simulink library "Yaw_Gearbox_Lib"  (R2025a)
settings: Solver=ode45  StartTime=0.0  StopTime=10.0  RelTol=1e-3  EnableMultiTasking=on
undefined symbols (not defined in the file): WT_Params
libraries: fl_lib x7, sdl_lib x4
Description:
  | Copyright 2009-2025 The MathWorks, Inc. MathWorks, Inc.
settings Model: Creator=smiller  LastModifiedBy=smiller
settings SolverCC: AlgebraicLoopSolver=TrustRegion
settings DataIOCC: LimitDataPoints=on  SaveFormat=Array  SignalLoggingSaveFormat=ModelDataLogs  ReturnWorkspaceOutputs=off
settings OptimizationCC: ReuseModelBlockBuffer=off  ExpressionDepthLimit=2147483647.0  LifeSpan=inf
settings DebuggingCC: UnderspecifiedInitializationDetection=Classic  MergeDetectMultiDrivingBlocksExec=none  SolverPrmCheckMsg=warning  FcnCallInpInsideContextMsg=warning  UnconnectedInputMsg=warning  UnconnectedOutputMsg=warning  UnconnectedLineMsg=warning  AllowSymbolicDim=off  StateNameClashWarn=warning  PregeneratedLibrarySubsystemCodeDiagnostic=none  SFUnexpectedBacktrackingDiag=warning  SFNoUnconditionalDefaultTransitionDiag=warning  SFExecutionAtInitializationDiag=none  ArithmeticOperatorsInVariantConditions=warning
settings HardwareCC: ProdBitPerPointer=32.0  ProdBitPerSizeT=32.0  ProdBitPerPtrDiffT=32.0  ProdLargestAtomicFloat=None  ProdIntDivRoundTo=Undefined  ProdEndianess=Unspecified  ProdWordSize=32.0  ProdHWDeviceType=32-bit Generic
settings ModelReferenceCC: EnableRefExpFcnMdlSchedulingChecks=on  PropagateSignalLabelsOutOfModel=off
settings SFSimCC: SimUseLocalCustomCode=off  CustomCodeUndefinedFunction=UseInterfaceOnly
settings RTWCC: RTWUseLocalCustomCode=off  GPUComputeCapability=3.5  DLArmComputeVersion=19.05
settings CodeAppCC: StateflowObjectComments=on
settings GRTTargetCC: TargetLangStandard=C89/C90 (ANSI)  CombineOutputUpdateFcns=off  GRTInterface=on
settings ConfigComp: CovMetricSettings=dw  CovSaveCumulativeToWorkspaceVar=on  CovSaveSingleToWorkspaceVar=on  CovExternalEMLEnable=off  CovSFcnEnable=off

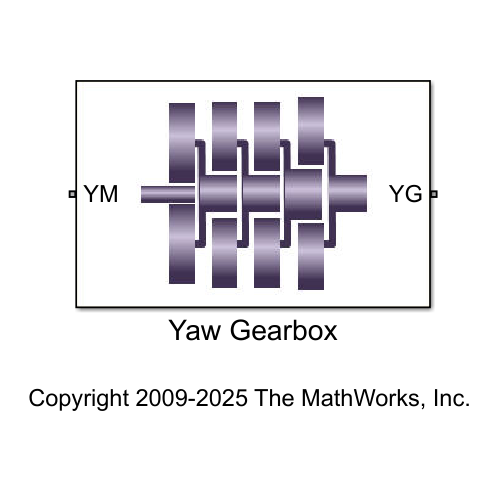
[thumbnail: Simulink's stored preview of the top-level diagram]
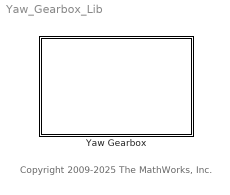
== system Yaw_Gearbox_Lib ==
  note: Copyright 2009-2025 The MathWorks, Inc.
  Yaw Gearbox : Subsystem
      mask Display: image('Yaw_Gearbox_IMAGE.jpg');

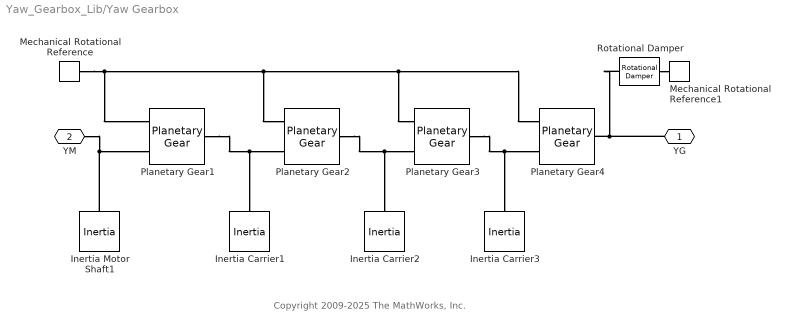
== system Yaw_Gearbox_Lib/Yaw Gearbox ==
  note: Copyright 2009-2025 The MathWorks, Inc.
  Inertia Carrier1 : fl_lib/Mechanical/Rotational Elements/Inertia  inertia=WT_Params.Yaw_Actuator.inertia_carrier kg*m^2  num_ports=foundation.enum.numPorts2.one  w_specify=on  w_priority=High  w=0 rad/s  w_nominal_specify=off  w_nominal_value=1  w_nominal_unit=rad/s  t_specify=off  t_priority=High  t=0 N*m  t_nominal_specify=off  t_nominal_value=1  t_nominal_unit=N*m
  Inertia Carrier2 : fl_lib/Mechanical/Rotational Elements/Inertia  inertia=WT_Params.Yaw_Actuator.inertia_carrier kg*m^2  num_ports=foundation.enum.numPorts2.one  w_specify=on  w_priority=High  w=0 rad/s  w_nominal_specify=off  w_nominal_value=1  w_nominal_unit=rad/s  t_specify=off  t_priority=High  t=0 N*m  t_nominal_specify=off  t_nominal_value=1  t_nominal_unit=N*m
  Inertia Carrier3 : fl_lib/Mechanical/Rotational Elements/Inertia  inertia=WT_Params.Yaw_Actuator.inertia_carrier kg*m^2  num_ports=foundation.enum.numPorts2.one  w_specify=on  w_priority=High  w=0 rad/s  w_nominal_specify=off  w_nominal_value=1  w_nominal_unit=rad/s  t_specify=off  t_priority=High  t=0 N*m  t_nominal_specify=off  t_nominal_value=1  t_nominal_unit=N*m
  Inertia Motor Shaft1 : fl_lib/Mechanical/Rotational Elements/Inertia  inertia=WT_Params.Yaw_Actuator.inertia_motor_shaft kg*m^2  num_ports=foundation.enum.numPorts2.one  w_specify=on  w_priority=High  w=0 rad/s  w_nominal_specify=off  w_nominal_value=1  w_nominal_unit=rad/s  t_specify=off  t_priority=High  t=0 N*m  t_nominal_specify=off  t_nominal_value=1  t_nominal_unit=N*m
  Mechanical Rotational Reference : fl_lib/Mechanical/Rotational Elements/Mechanical Rotational Reference
  Mechanical Rotational Reference1 : fl_lib/Mechanical/Rotational Elements/Mechanical Rotational Reference
  Planetary Gear1 : sdl_lib/Gears/Planetary Gear  rs_ratio=WT_Params.Yaw_Actuator.p_gear_rato_step_1-1  friction_model=1  efficiency=[ 0.96 0.98 ]  temperature_TLU=[ 280 300 320 ] K  efficiency_sp_TLU=[ 0.95 0.9 0.85 ]  efficiency_rp_TLU=[ 0.95 0.9 0.85 ]  pwr_thr=[ 0.001 0.001 ] W  mu_visc=[ 0 0 ] N*m/(rad/s)  model_inertia=0  sun_inertia=1e-10 kg*m^2  ring_inertia=1e-10 kg*m^2  carrier_inertia=1e-10 kg*m^2  carrier_radius=0.01 m  planet_inertia=0.001 kg*m^2  planet_mass=1e-10 kg  thermal_mass=50 J/K  T_init=300 K
  Planetary Gear2 : sdl_lib/Gears/Planetary Gear  rs_ratio=WT_Params.Yaw_Actuator.p_gear_rato_step_2-1  friction_model=1  efficiency=[ 0.96 0.98 ]  temperature_TLU=[ 280 300 320 ] K  efficiency_sp_TLU=[ 0.95 0.9 0.85 ]  efficiency_rp_TLU=[ 0.95 0.9 0.85 ]  pwr_thr=[ 0.001 0.001 ] W  mu_visc=[ 0 0 ] N*m/(rad/s)  model_inertia=0  sun_inertia=1e-10 kg*m^2  ring_inertia=1e-10 kg*m^2  carrier_inertia=1e-10 kg*m^2  carrier_radius=0.01 m  planet_inertia=0.001 kg*m^2  planet_mass=1e-10 kg  thermal_mass=50 J/K  T_init=300 K
  Planetary Gear3 : sdl_lib/Gears/Planetary Gear  rs_ratio=WT_Params.Yaw_Actuator.p_gear_rato_step_3-1  friction_model=1  efficiency=[ 0.96 0.98 ]  temperature_TLU=[ 280 300 320 ] K  efficiency_sp_TLU=[ 0.95 0.9 0.85 ]  efficiency_rp_TLU=[ 0.95 0.9 0.85 ]  pwr_thr=[ 0.001 0.001 ] W  mu_visc=[ 0 0 ] N*m/(rad/s)  model_inertia=0  sun_inertia=1e-10 kg*m^2  ring_inertia=1e-10 kg*m^2  carrier_inertia=1e-10 kg*m^2  carrier_radius=0.01 m  planet_inertia=0.001 kg*m^2  planet_mass=1e-10 kg  thermal_mass=50 J/K  T_init=300 K
  Planetary Gear4 : sdl_lib/Gears/Planetary Gear  rs_ratio=WT_Params.Yaw_Actuator.p_gear_rato_step_4-1  friction_model=1  efficiency=[ 0.96 0.98 ]  temperature_TLU=[ 280 300 320 ] K  efficiency_sp_TLU=[ 0.95 0.9 0.85 ]  efficiency_rp_TLU=[ 0.95 0.9 0.85 ]  pwr_thr=[ 0.001 0.001 ] W  mu_visc=[ 0 0 ] N*m/(rad/s)  model_inertia=0  sun_inertia=1e-10 kg*m^2  ring_inertia=1e-10 kg*m^2  carrier_inertia=1e-10 kg*m^2  carrier_radius=0.01 m  planet_inertia=0.001 kg*m^2  planet_mass=1e-10 kg  thermal_mass=50 J/K  T_init=300 K
  Rotational Damper : fl_lib/Mechanical/Rotational Elements/Rotational Damper  D=WT_Params.Yaw_Actuator.damping N*m/(rad/s)  w_specify=off  w_priority=High  w=0 rad/s  w_nominal_specify=off  w_nominal_value=1  w_nominal_unit=rad/s  t_specify=off  t_priority=High  t=0 N*m  t_nominal_specify=off  t_nominal_value=1  t_nominal_unit=N*m
  YG : PMIOPort  Side=Right
  YM : PMIOPort  Port=2  Side=Left
  connections:
  Planetary Gear1/LConn1 -- Planetary Gear2/RConn2 -- Inertia Carrier1/LConn1
  Planetary Gear2/LConn1 -- Planetary Gear3/RConn2 -- Inertia Carrier2/LConn1
  Planetary Gear3/LConn1 -- Planetary Gear4/RConn2 -- Inertia Carrier3/LConn1
  Mechanical Rotational Reference/LConn1 -- Planetary Gear1/RConn1 -- Planetary Gear2/RConn1 -- Planetary Gear3/RConn1 -- Planetary Gear4/RConn1
  Inertia Motor Shaft1/LConn1 -- Planetary Gear1/RConn2 -- YM/RConn1
  Rotational Damper/LConn1 -- YG/RConn1 -- Planetary Gear4/LConn1
  Rotational Damper/RConn1 -- Mechanical Rotational Reference1/LConn1
